simulink model "rehab_arm_3dof"  (R2025a)
settings: Solver=ode4  StartTime=0.0  StopTime=Tsim  FixedStep=Ts  RelTol=1e-3
values from neighbouring files (symbols this model uses):
  Pt = Pt(:);\n'      'td = zeros(3,1);\n'      'for i = 1:size(dist,1)\n'      '    j = round(dist(i,3));\n'      '    if t >= dist(i,1) && t < dist(i,2) && j >= 1 && j <= 3\n'      '        td(j) = td(j) + dist(i,4);\n'      '    end\n'      'end\n'      'rhs = tau(:) + td - arm_C(q, qd, Pt)*qd - arm_G(q, Pt) - Bv(:).*qd;\n'      'qdd = arm_M(q, Pt) \\ rhs;\n']))    [build_rehab_arm_model.m]
  q0 = deg2rad([30; 60; 45])    [validate_simscape.m]
undefined symbols (not defined in the file or in its folder): Bv, dist, Kd, Ki, Kp, noise_q, noise_qd, Pm, tau_max, Ts
settings Model: Creator=anant  LastModifiedBy=anant
settings DataIOCC: SaveOutput=off  SignalLogging=off  SaveTime=off

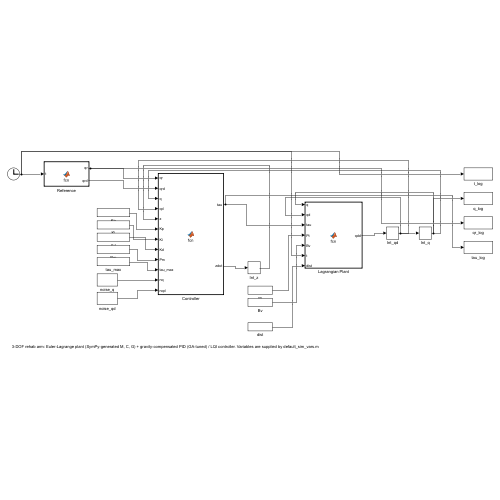
[thumbnail: Simulink's stored preview of the top-level diagram]
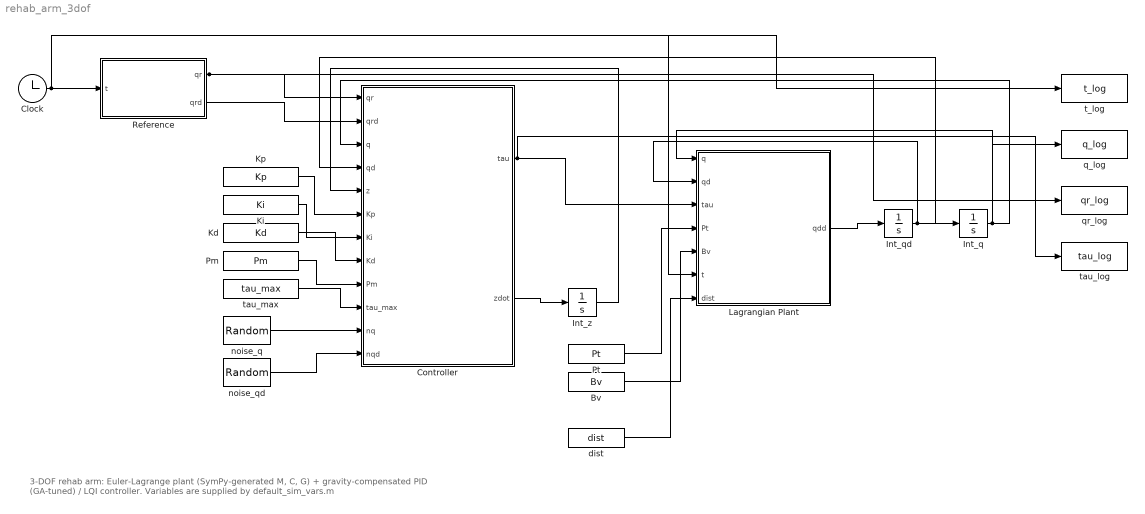
== system rehab_arm_3dof ==
  note: 3-DOF rehab arm: Euler-Lagrange plant (SymPy-generated M, C, G) + gravity-compensated PID (GA-tuned) / LQI controller. Variables are supplied by default_sim_vars.m
  Bv : Constant  Value=Bv  VectorParams1D=off
  Clock : Clock
  Controller : MATLAB Function  TreatAsAtomicUnit=on
  Int_q : Integrator  InitialCondition=q0
  Int_qd : Integrator  InitialCondition=zeros(3,1)
  Int_z : Integrator  InitialCondition=zeros(3,1)
  Kd : Constant  Value=Kd  VectorParams1D=off
  Ki : Constant  Value=Ki  VectorParams1D=off
  Kp : Constant  Value=Kp  VectorParams1D=off
  Lagrangian Plant : MATLAB Function  TreatAsAtomicUnit=on
  Pm : Constant  Value=Pm  VectorParams1D=off
  Pt : Constant  Value=Pt  VectorParams1D=off
  Reference : MATLAB Function  TreatAsAtomicUnit=on
  dist : Constant  Value=dist  VectorParams1D=off
  noise_q : RandomNumber  Variance=noise_q^2*ones(3,1)  Seed=[11 12 13]  SampleTime=Ts
  noise_qd : RandomNumber  Variance=noise_qd^2*ones(3,1)  Seed=[21 22 23]  SampleTime=Ts
  q_log : ToWorkspace  VariableName=q_log  SampleTime=-1
  qr_log : ToWorkspace  VariableName=qr_log  SampleTime=-1
  t_log : ToWorkspace  VariableName=t_log  SampleTime=-1
  tau_log : ToWorkspace  VariableName=tau_log  SampleTime=-1
  tau_max : Constant  Value=tau_max  VectorParams1D=off
  wires:
  Clock/1 -> Reference/1(t), Lagrangian Plant/6(t), t_log/1
  Reference/1(qr) -> Controller/1(qr), qr_log/1
  Reference/2(qrd) -> Controller/2(qrd)
  Int_q/1 -> Controller/3(q), Lagrangian Plant/1(q), q_log/1
  Int_qd/1 -> Controller/4(qd), Lagrangian Plant/2(qd), Int_q/1
  Int_z/1 -> Controller/5(z)
  Kp/1 -> Controller/6(Kp)
  Ki/1 -> Controller/7(Ki)
  Kd/1 -> Controller/8(Kd)
  Pm/1 -> Controller/9(Pm)
  tau_max/1 -> Controller/10(tau_max)
  noise_q/1 -> Controller/11(nq)
  noise_qd/1 -> Controller/12(nqd)
  Controller/2(zdot) -> Int_z/1
  Controller/1(tau) -> Lagrangian Plant/3(tau), tau_log/1
  Pt/1 -> Lagrangian Plant/4(Pt)
  Bv/1 -> Lagrangian Plant/5(Bv)
  dist/1 -> Lagrangian Plant/7(dist)
  Lagrangian Plant/1(qdd) -> Int_qd/1

== matlab function rehab_arm_3dof/Controller ==
  data: qr input; tau output; qrd input; q input; qd input; z input; Kp input; Ki input; Kd input; Pm input; tau_max input; nq input; nqd input; zdot output
function [tau, zdot] = fcn(qr, qrd, q, qd, z, Kp, Ki, Kd, Pm, tau_max, nq, nqd)
% Gravity-compensated PID / LQI with saturation + conditional-integration anti-windup
qm  = q(:)  + nq(:);      % encoder noise
qdm = qd(:) + nqd(:);     % velocity-estimate noise
e   = qr(:)  - qm;
ed  = qrd(:) - qdm;
tau_u = arm_G(qm, Pm(:)) + Kp*e + Ki*z(:) + Kd*ed;
tau = min(max(tau_u, -tau_max(:)), tau_max(:));
zdot = e .* double(abs(tau_u) <= tau_max(:));

== matlab function rehab_arm_3dof/Reference ==
  data: t input; qr output; qrd output
function [qr, qrd] = fcn(t)
% min-jerk rehab task (rehab_task.m)
[qr, qrd, ~] = rehab_task(t);

== matlab function rehab_arm_3dof/Lagrangian Plant ==
  data: q input; qdd output; qd input; tau input; Pt input; Bv input; t input; dist input
function qdd = fcn(q, qd, tau, Pt, Bv, t, dist)
% Euler-Lagrange forward dynamics of the TRUE arm (may differ from model Pm)
q = q(:); qd = qd(:); Pt = Pt(:);
td = zeros(3,1);
for i = 1:size(dist,1)
    j = round(dist(i,3));
    if t >= dist(i,1) && t < dist(i,2) && j >= 1 && j <= 3
        td(j) = td(j) + dist(i,4);
    end
end
rhs = tau(:) + td - arm_C(q, qd, Pt)*qd - arm_G(q, Pt) - Bv(:).*qd;
qdd = arm_M(q, Pt) \ rhs;
